simulink model "solar_pv_protected_c07_circuit"  (R2026b)
settings: Solver=VariableStepAuto
model workspace (MAT data in the model file):
  candidate_owner = 'pv_protection_integration_20261023_r01'
  solar_edit_metadata : object (value not decoded)
libraries: fl_lib x149, ee_lib x16, ltc4364demo_lib x3, batteryecm_lib x1, solarprotect_lib x1
(part 15 of 16)

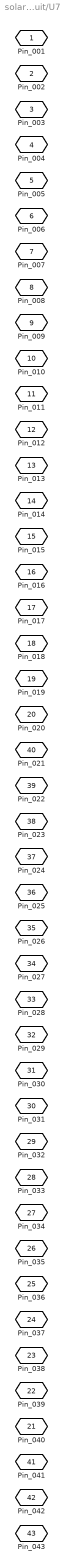
== system solar_pv_protected_c07_circuit/U7 ==
  Pin_001 : PMIOPort  Description=|  Side=Left  ConnectionType=Connection: foundation.electrical.electrical
      | 識別名　　　　　　　; Pin_001
      | 種別　　　　　　　　; Simscape Connection Port（階層境界の物理端子）
      | 所属部品　　　　　　; U7
      | 配置目的　　　　　　; 内部の電気ノードを、この外箱の外側の対応端子へ引き出す。
      | 対応端子　　　　　　; lconn:1／1番 GP0
      | 接続ラベル　　　　　; ラベルなし。接続は実線と境界対応で定義する。
      | モデルの範囲　　　　; 実部品を1個追加する表現ではない。端子自体に増幅・遮断・測定機能を持たない。
      | 端子番号の注意　　　; Connection Portの番号は外箱内の対応番号であり、実パッケージのピン番号とは区別する。
      | 確認の範囲　　　　　; 実ポートと階層対応による静的接続の説明。電気特性の再現性は所属部品の説明を参照する。
      | 
      | 従来の補足　　　　　; 以前のDescriptionを以下に保持する。
      | Physical U7 pin 1 / GP0
      | 
      | 【この説明欄の略語・記号】
      | 用語1　　　　　　　 ; GPIO：General-Purpose Input/Output（汎用入出力端子）。入力・出力や周辺機能に割り当てられる端子。GPの後の数字はRP2040の端子信号番号で、基板上の物理ピン番号とは別。
  Pin_002 : PMIOPort  Description=|  Port=2  Side=Left  ConnectionType=Connection: foundation.electrical.electrical
      | 識別名　　　　　　　; Pin_002
      | 種別　　　　　　　　; Simscape Connection Port（階層境界の物理端子）
      | 所属部品　　　　　　; U7
      | 配置目的　　　　　　; 内部の電気ノードを、この外箱の外側の対応端子へ引き出す。
      | 対応端子　　　　　　; lconn:2／2番 GP1
      | 接続ラベル　　　　　; ラベルなし。接続は実線と境界対応で定義する。
      | モデルの範囲　　　　; 実部品を1個追加する表現ではない。端子自体に増幅・遮断・測定機能を持たない。
      | 端子番号の注意　　　; Connection Portの番号は外箱内の対応番号であり、実パッケージのピン番号とは区別する。
      | 確認の範囲　　　　　; 実ポートと階層対応による静的接続の説明。電気特性の再現性は所属部品の説明を参照する。
      | 
      | 従来の補足　　　　　; 以前のDescriptionを以下に保持する。
      | Physical U7 pin 2 / GP1
      | 
      | 【この説明欄の略語・記号】
      | 用語1　　　　　　　 ; GPIO：General-Purpose Input/Output（汎用入出力端子）。入力・出力や周辺機能に割り当てられる端子。GPの後の数字はRP2040の端子信号番号で、基板上の物理ピン番号とは別。
  Pin_003 : PMIOPort  Description=|  Port=3  Side=Left  ConnectionType=Connection: foundation.electrical.electrical
      | 識別名　　　　　　　; Pin_003
      | 種別　　　　　　　　; Simscape Connection Port（階層境界の物理端子）
      | 所属部品　　　　　　; U7
      | 配置目的　　　　　　; 内部の電気ノードを、この外箱の外側の対応端子へ引き出す。
      | 対応端子　　　　　　; lconn:3／3番 GND
      | 接続ラベル　　　　　; GND、PROT_RETURN
      | モデルの範囲　　　　; 実部品を1個追加する表現ではない。端子自体に増幅・遮断・測定機能を持たない。
      | 端子番号の注意　　　; Connection Portの番号は外箱内の対応番号であり、実パッケージのピン番号とは区別する。
      | 確認の範囲　　　　　; 実ポートと階層対応による静的接続の説明。電気特性の再現性は所属部品の説明を参照する。
      | 
      | 従来の補足　　　　　; 以前のDescriptionを以下に保持する。
      | Physical U7 pin 3 / GND
      | 
      | 【この説明欄の略語・記号】
      | 用語1　　　　　　　 ; GND：Ground（回路の基準電位・電流帰路）。この図の共通基準。保護接地や大地への接続を意味するとは限らない。
      | 用語2　　　　　　　 ; PROT_RETURN：保護回路の共通帰路。PROTはProtection（保護）、RETURNは帰路。プロトタイプの略ではなく、現回路では共通GNDへつながる。
  Pin_004 : PMIOPort  Description=|  Port=4  Side=Left  ConnectionType=Connection: foundation.electrical.electrical
      | 識別名　　　　　　　; Pin_004
      | 種別　　　　　　　　; Simscape Connection Port（階層境界の物理端子）
      | 所属部品　　　　　　; U7
      | 配置目的　　　　　　; 内部の電気ノードを、この外箱の外側の対応端子へ引き出す。
      | 対応端子　　　　　　; lconn:4／4番 GP2
      | 接続ラベル　　　　　; ラベルなし。接続は実線と境界対応で定義する。
      | モデルの範囲　　　　; 実部品を1個追加する表現ではない。端子自体に増幅・遮断・測定機能を持たない。
      | 端子番号の注意　　　; Connection Portの番号は外箱内の対応番号であり、実パッケージのピン番号とは区別する。
      | 確認の範囲　　　　　; 実ポートと階層対応による静的接続の説明。電気特性の再現性は所属部品の説明を参照する。
      | 
      | 従来の補足　　　　　; 以前のDescriptionを以下に保持する。
      | Physical U7 pin 4 / GP2
      | 
      | 【この説明欄の略語・記号】
      | 用語1　　　　　　　 ; GPIO：General-Purpose Input/Output（汎用入出力端子）。入力・出力や周辺機能に割り当てられる端子。GPの後の数字はRP2040の端子信号番号で、基板上の物理ピン番号とは別。
  Pin_005 : PMIOPort  Description=|  Port=5  Side=Left  ConnectionType=Connection: foundation.electrical.electrical
      | 識別名　　　　　　　; Pin_005
      | 種別　　　　　　　　; Simscape Connection Port（階層境界の物理端子）
      | 所属部品　　　　　　; U7
      | 配置目的　　　　　　; 内部の電気ノードを、この外箱の外側の対応端子へ引き出す。
      | 対応端子　　　　　　; lconn:5／5番 GP3
      | 接続ラベル　　　　　; ラベルなし。接続は実線と境界対応で定義する。
      | モデルの範囲　　　　; 実部品を1個追加する表現ではない。端子自体に増幅・遮断・測定機能を持たない。
      | 端子番号の注意　　　; Connection Portの番号は外箱内の対応番号であり、実パッケージのピン番号とは区別する。
      | 確認の範囲　　　　　; 実ポートと階層対応による静的接続の説明。電気特性の再現性は所属部品の説明を参照する。
      | 
      | 従来の補足　　　　　; 以前のDescriptionを以下に保持する。
      | Physical U7 pin 5 / GP3
      | 
      | 【この説明欄の略語・記号】
      | 用語1　　　　　　　 ; GPIO：General-Purpose Input/Output（汎用入出力端子）。入力・出力や周辺機能に割り当てられる端子。GPの後の数字はRP2040の端子信号番号で、基板上の物理ピン番号とは別。
  Pin_006 : PMIOPort  Description=|  Port=6  Side=Left  ConnectionType=Connection: foundation.electrical.electrical
      | 識別名　　　　　　　; Pin_006
      | 種別　　　　　　　　; Simscape Connection Port（階層境界の物理端子）
      | 所属部品　　　　　　; U7
      | 配置目的　　　　　　; 内部の電気ノードを、この外箱の外側の対応端子へ引き出す。
      | 対応端子　　　　　　; lconn:6／6番 GP4
      | 接続ラベル　　　　　; ラベルなし。接続は実線と境界対応で定義する。
      | モデルの範囲　　　　; 実部品を1個追加する表現ではない。端子自体に増幅・遮断・測定機能を持たない。
      | 端子番号の注意　　　; Connection Portの番号は外箱内の対応番号であり、実パッケージのピン番号とは区別する。
      | 確認の範囲　　　　　; 実ポートと階層対応による静的接続の説明。電気特性の再現性は所属部品の説明を参照する。
      | 
      | 従来の補足　　　　　; 以前のDescriptionを以下に保持する。
      | Physical U7 pin 6 / GP4
      | 
      | 【この説明欄の略語・記号】
      | 用語1　　　　　　　 ; GPIO：General-Purpose Input/Output（汎用入出力端子）。入力・出力や周辺機能に割り当てられる端子。GPの後の数字はRP2040の端子信号番号で、基板上の物理ピン番号とは別。
  Pin_007 : PMIOPort  Description=|  Port=7  Side=Left  ConnectionType=Connection: foundation.electrical.electrical
      | 識別名　　　　　　　; Pin_007
      | 種別　　　　　　　　; Simscape Connection Port（階層境界の物理端子）
      | 所属部品　　　　　　; U7
      | 配置目的　　　　　　; 内部の電気ノードを、この外箱の外側の対応端子へ引き出す。
      | 対応端子　　　　　　; lconn:7／7番 GP5
      | 接続ラベル　　　　　; ラベルなし。接続は実線と境界対応で定義する。
      | モデルの範囲　　　　; 実部品を1個追加する表現ではない。端子自体に増幅・遮断・測定機能を持たない。
      | 端子番号の注意　　　; Connection Portの番号は外箱内の対応番号であり、実パッケージのピン番号とは区別する。
      | 確認の範囲　　　　　; 実ポートと階層対応による静的接続の説明。電気特性の再現性は所属部品の説明を参照する。
      | 
      | 従来の補足　　　　　; 以前のDescriptionを以下に保持する。
      | Physical U7 pin 7 / GP5
      | 
      | 【この説明欄の略語・記号】
      | 用語1　　　　　　　 ; GPIO：General-Purpose Input/Output（汎用入出力端子）。入力・出力や周辺機能に割り当てられる端子。GPの後の数字はRP2040の端子信号番号で、基板上の物理ピン番号とは別。
  Pin_008 : PMIOPort  Description=|  Port=8  Side=Left  ConnectionType=Connection: foundation.electrical.electrical
      | 識別名　　　　　　　; Pin_008
      | 種別　　　　　　　　; Simscape Connection Port（階層境界の物理端子）
      | 所属部品　　　　　　; U7
      | 配置目的　　　　　　; 内部の電気ノードを、この外箱の外側の対応端子へ引き出す。
      | 対応端子　　　　　　; lconn:8／8番 GND
      | 接続ラベル　　　　　; GND、PROT_RETURN
      | モデルの範囲　　　　; 実部品を1個追加する表現ではない。端子自体に増幅・遮断・測定機能を持たない。
      | 端子番号の注意　　　; Connection Portの番号は外箱内の対応番号であり、実パッケージのピン番号とは区別する。
      | 確認の範囲　　　　　; 実ポートと階層対応による静的接続の説明。電気特性の再現性は所属部品の説明を参照する。
      | 
      | 従来の補足　　　　　; 以前のDescriptionを以下に保持する。
      | Physical U7 pin 8 / GND
      | 
      | 【この説明欄の略語・記号】
      | 用語1　　　　　　　 ; GND：Ground（回路の基準電位・電流帰路）。この図の共通基準。保護接地や大地への接続を意味するとは限らない。
      | 用語2　　　　　　　 ; PROT_RETURN：保護回路の共通帰路。PROTはProtection（保護）、RETURNは帰路。プロトタイプの略ではなく、現回路では共通GNDへつながる。
  Pin_009 : PMIOPort  Description=|  Port=9  Side=Left  ConnectionType=Connection: foundation.electrical.electrical
      | 識別名　　　　　　　; Pin_009
      | 種別　　　　　　　　; Simscape Connection Port（階層境界の物理端子）
      | 所属部品　　　　　　; U7
      | 配置目的　　　　　　; 内部の電気ノードを、この外箱の外側の対応端子へ引き出す。
      | 対応端子　　　　　　; lconn:9／9番 GP6
      | 接続ラベル　　　　　; GP6
      | モデルの範囲　　　　; 実部品を1個追加する表現ではない。端子自体に増幅・遮断・測定機能を持たない。
      | 端子番号の注意　　　; Connection Portの番号は外箱内の対応番号であり、実パッケージのピン番号とは区別する。
      | 確認の範囲　　　　　; 実ポートと階層対応による静的接続の説明。電気特性の再現性は所属部品の説明を参照する。
      | 
      | 従来の補足　　　　　; 以前のDescriptionを以下に保持する。
      | Physical U7 pin 9 / GP6
      | 
      | 【この説明欄の略語・記号】
      | 用語1　　　　　　　 ; GPIO：General-Purpose Input/Output（汎用入出力端子）。入力・出力や周辺機能に割り当てられる端子。GPの後の数字はRP2040の端子信号番号で、基板上の物理ピン番号とは別。
  Pin_010 : PMIOPort  Description=|  Port=10  Side=Left  ConnectionType=Connection: foundation.electrical.electrical
      | 識別名　　　　　　　; Pin_010
      | 種別　　　　　　　　; Simscape Connection Port（階層境界の物理端子）
      | 所属部品　　　　　　; U7
      | 配置目的　　　　　　; 内部の電気ノードを、この外箱の外側の対応端子へ引き出す。
      | 対応端子　　　　　　; lconn:10／10番 GP7
      | 接続ラベル　　　　　; GP7
      | モデルの範囲　　　　; 実部品を1個追加する表現ではない。端子自体に増幅・遮断・測定機能を持たない。
      | 端子番号の注意　　　; Connection Portの番号は外箱内の対応番号であり、実パッケージのピン番号とは区別する。
      | 確認の範囲　　　　　; 実ポートと階層対応による静的接続の説明。電気特性の再現性は所属部品の説明を参照する。
      | 
      | 従来の補足　　　　　; 以前のDescriptionを以下に保持する。
      | Physical U7 pin 10 / GP7
      | 
      | 【この説明欄の略語・記号】
      | 用語1　　　　　　　 ; GPIO：General-Purpose Input/Output（汎用入出力端子）。入力・出力や周辺機能に割り当てられる端子。GPの後の数字はRP2040の端子信号番号で、基板上の物理ピン番号とは別。
  Pin_011 : PMIOPort  Description=|  Port=11  Side=Left  ConnectionType=Connection: foundation.electrical.electrical
      | 識別名　　　　　　　; Pin_011
      | 種別　　　　　　　　; Simscape Connection Port（階層境界の物理端子）
      | 所属部品　　　　　　; U7
      | 配置目的　　　　　　; 内部の電気ノードを、この外箱の外側の対応端子へ引き出す。
      | 対応端子　　　　　　; lconn:11／11番 GP8
      | 接続ラベル　　　　　; BIAS_EN
      | モデルの範囲　　　　; 実部品を1個追加する表現ではない。端子自体に増幅・遮断・測定機能を持たない。
      | 端子番号の注意　　　; Connection Portの番号は外箱内の対応番号であり、実パッケージのピン番号とは区別する。
      | 確認の範囲　　　　　; 実ポートと階層対応による静的接続の説明。電気特性の再現性は所属部品の説明を参照する。
      | 
      | 従来の補足　　　　　; 以前のDescriptionを以下に保持する。
      | Physical U7 pin 11 / GP8
      | 
      | 【この説明欄の略語・記号】
      | 用語1　　　　　　　 ; GPIO：General-Purpose Input/Output（汎用入出力端子）。入力・出力や周辺機能に割り当てられる端子。GPの後の数字はRP2040の端子信号番号で、基板上の物理ピン番号とは別。
      | 用語2　　　　　　　 ; EN：Enable（動作許可）。対象機能の動作を許可する信号。端子ごとの有効レベルや接続状態に従う。
  Pin_012 : PMIOPort  Description=|  Port=12  Side=Left  ConnectionType=Connection: foundation.electrical.electrical
      | 識別名　　　　　　　; Pin_012
      | 種別　　　　　　　　; Simscape Connection Port（階層境界の物理端子）
      | 所属部品　　　　　　; U7
      | 配置目的　　　　　　; 内部の電気ノードを、この外箱の外側の対応端子へ引き出す。
      | 対応端子　　　　　　; lconn:12／12番 GP9
      | 接続ラベル　　　　　; BIAS_PG
      | モデルの範囲　　　　; 実部品を1個追加する表現ではない。端子自体に増幅・遮断・測定機能を持たない。
      | 端子番号の注意　　　; Connection Portの番号は外箱内の対応番号であり、実パッケージのピン番号とは区別する。
      | 確認の範囲　　　　　; 実ポートと階層対応による静的接続の説明。電気特性の再現性は所属部品の説明を参照する。
      | 
      | 従来の補足　　　　　; 以前のDescriptionを以下に保持する。
      | Physical U7 pin 12 / GP9
      | 
      | 【この説明欄の略語・記号】
      | 用語1　　　　　　　 ; IC：Integrated Circuit（集積回路）。複数の電子素子と機能を小さな半導体チップに集積した部品。
      | 用語2　　　　　　　 ; GPIO：General-Purpose Input/Output（汎用入出力端子）。入力・出力や周辺機能に割り当てられる端子。GPの後の数字はRP2040の端子信号番号で、基板上の物理ピン番号とは別。
      | 用語3　　　　　　　 ; PG：Power Good（電源状態通知）。電源出力が規定状態にあるかを知らせる信号。プルアップ条件と実際の通知条件は対象ICの説明で確認する。
  Pin_013 : PMIOPort  Description=|  Port=13  Side=Left  ConnectionType=Connection: foundation.electrical.electrical
      | 識別名　　　　　　　; Pin_013
      | 種別　　　　　　　　; Simscape Connection Port（階層境界の物理端子）
      | 所属部品　　　　　　; U7
      | 配置目的　　　　　　; 内部の電気ノードを、この外箱の外側の対応端子へ引き出す。
      | 対応端子　　　　　　; lconn:13／13番 GND
      | 接続ラベル　　　　　; GND、PROT_RETURN
      | モデルの範囲　　　　; 実部品を1個追加する表現ではない。端子自体に増幅・遮断・測定機能を持たない。
      | 端子番号の注意　　　; Connection Portの番号は外箱内の対応番号であり、実パッケージのピン番号とは区別する。
      | 確認の範囲　　　　　; 実ポートと階層対応による静的接続の説明。電気特性の再現性は所属部品の説明を参照する。
      | 
      | 従来の補足　　　　　; 以前のDescriptionを以下に保持する。
      | Physical U7 pin 13 / GND
      | 
      | 【この説明欄の略語・記号】
      | 用語1　　　　　　　 ; GND：Ground（回路の基準電位・電流帰路）。この図の共通基準。保護接地や大地への接続を意味するとは限らない。
      | 用語2　　　　　　　 ; PROT_RETURN：保護回路の共通帰路。PROTはProtection（保護）、RETURNは帰路。プロトタイプの略ではなく、現回路では共通GNDへつながる。
  Pin_014 : PMIOPort  Description=|  Port=14  Side=Left  ConnectionType=Connection: foundation.electrical.electrical
      | 識別名　　　　　　　; Pin_014
      | 種別　　　　　　　　; Simscape Connection Port（階層境界の物理端子）
      | 所属部品　　　　　　; U7
      | 配置目的　　　　　　; 内部の電気ノードを、この外箱の外側の対応端子へ引き出す。
      | 対応端子　　　　　　; lconn:14／14番 GP10
      | 接続ラベル　　　　　; ラベルなし。接続は実線と境界対応で定義する。
      | モデルの範囲　　　　; 実部品を1個追加する表現ではない。端子自体に増幅・遮断・測定機能を持たない。
      | 端子番号の注意　　　; Connection Portの番号は外箱内の対応番号であり、実パッケージのピン番号とは区別する。
      | 確認の範囲　　　　　; 実ポートと階層対応による静的接続の説明。電気特性の再現性は所属部品の説明を参照する。
      | 
      | 従来の補足　　　　　; 以前のDescriptionを以下に保持する。
      | Physical U7 pin 14 / GP10
      | 
      | 【この説明欄の略語・記号】
      | 用語1　　　　　　　 ; GPIO：General-Purpose Input/Output（汎用入出力端子）。入力・出力や周辺機能に割り当てられる端子。GPの後の数字はRP2040の端子信号番号で、基板上の物理ピン番号とは別。
  Pin_015 : PMIOPort  Description=|  Port=15  Side=Left  ConnectionType=Connection: foundation.electrical.electrical
      | 識別名　　　　　　　; Pin_015
      | 種別　　　　　　　　; Simscape Connection Port（階層境界の物理端子）
      | 所属部品　　　　　　; U7
      | 配置目的　　　　　　; 内部の電気ノードを、この外箱の外側の対応端子へ引き出す。
      | 対応端子　　　　　　; lconn:15／15番 GP11
      | 接続ラベル　　　　　; MAIN_EN
      | モデルの範囲　　　　; 実部品を1個追加する表現ではない。端子自体に増幅・遮断・測定機能を持たない。
      | 端子番号の注意　　　; Connection Portの番号は外箱内の対応番号であり、実パッケージのピン番号とは区別する。
      | 確認の範囲　　　　　; 実ポートと階層対応による静的接続の説明。電気特性の再現性は所属部品の説明を参照する。
      | 
      | 従来の補足　　　　　; 以前のDescriptionを以下に保持する。
      | Physical U7 pin 15 / GP11
      | 
      | 【この説明欄の略語・記号】
      | 用語1　　　　　　　 ; GPIO：General-Purpose Input/Output（汎用入出力端子）。入力・出力や周辺機能に割り当てられる端子。GPの後の数字はRP2040の端子信号番号で、基板上の物理ピン番号とは別。
      | 用語2　　　　　　　 ; EN：Enable（動作許可）。対象機能の動作を許可する信号。端子ごとの有効レベルや接続状態に従う。
  Pin_016 : PMIOPort  Description=|  Port=16  Side=Left  ConnectionType=Connection: foundation.electrical.electrical
      | 識別名　　　　　　　; Pin_016
      | 種別　　　　　　　　; Simscape Connection Port（階層境界の物理端子）
      | 所属部品　　　　　　; U7
      | 配置目的　　　　　　; 内部の電気ノードを、この外箱の外側の対応端子へ引き出す。
      | 対応端子　　　　　　; lconn:16／16番 GP12
      | 接続ラベル　　　　　; ラベルなし。接続は実線と境界対応で定義する。
      | モデルの範囲　　　　; 実部品を1個追加する表現ではない。端子自体に増幅・遮断・測定機能を持たない。
      | 端子番号の注意　　　; Connection Portの番号は外箱内の対応番号であり、実パッケージのピン番号とは区別する。
      | 確認の範囲　　　　　; 実ポートと階層対応による静的接続の説明。電気特性の再現性は所属部品の説明を参照する。
      | 
      | 従来の補足　　　　　; 以前のDescriptionを以下に保持する。
      | Physical U7 pin 16 / GP12
      | 
      | 【この説明欄の略語・記号】
      | 用語1　　　　　　　 ; GPIO：General-Purpose Input/Output（汎用入出力端子）。入力・出力や周辺機能に割り当てられる端子。GPの後の数字はRP2040の端子信号番号で、基板上の物理ピン番号とは別。
  Pin_017 : PMIOPort  Description=|  Port=17  Side=Left  ConnectionType=Connection: foundation.electrical.electrical
      | 識別名　　　　　　　; Pin_017
      | 種別　　　　　　　　; Simscape Connection Port（階層境界の物理端子）
      | 所属部品　　　　　　; U7
      | 配置目的　　　　　　; 内部の電気ノードを、この外箱の外側の対応端子へ引き出す。
      | 対応端子　　　　　　; lconn:17／17番 GP13
      | 接続ラベル　　　　　; PROTECTION_FLT_N
      | モデルの範囲　　　　; 実部品を1個追加する表現ではない。端子自体に増幅・遮断・測定機能を持たない。
      | 端子番号の注意　　　; Connection Portの番号は外箱内の対応番号であり、実パッケージのピン番号とは区別する。
      | 確認の範囲　　　　　; 実ポートと階層対応による静的接続の説明。電気特性の再現性は所属部品の説明を参照する。
      | 
      | 従来の補足　　　　　; 以前のDescriptionを以下に保持する。
      | Physical U7 pin 17 / GP13
      | 
      | 【この説明欄の略語・記号】
      | 用語1　　　　　　　 ; GPIO：General-Purpose Input/Output（汎用入出力端子）。入力・出力や周辺機能に割り当てられる端子。GPの後の数字はRP2040の端子信号番号で、基板上の物理ピン番号とは別。
      | 用語2　　　　　　　 ; FLT：Fault（故障状態通知）。LTC4364の故障警告出力。全種類の異常や逆流を一律に通知する信号という意味ではない。
  Pin_018 : PMIOPort  Description=|  Port=18  Side=Left  ConnectionType=Connection: foundation.electrical.electrical
      | 識別名　　　　　　　; Pin_018
      | 種別　　　　　　　　; Simscape Connection Port（階層境界の物理端子）
      | 所属部品　　　　　　; U7
      | 配置目的　　　　　　; 内部の電気ノードを、この外箱の外側の対応端子へ引き出す。
      | 対応端子　　　　　　; lconn:18／18番 GND
      | 接続ラベル　　　　　; GND、PROT_RETURN
      | モデルの範囲　　　　; 実部品を1個追加する表現ではない。端子自体に増幅・遮断・測定機能を持たない。
      | 端子番号の注意　　　; Connection Portの番号は外箱内の対応番号であり、実パッケージのピン番号とは区別する。
      | 確認の範囲　　　　　; 実ポートと階層対応による静的接続の説明。電気特性の再現性は所属部品の説明を参照する。
      | 
      | 従来の補足　　　　　; 以前のDescriptionを以下に保持する。
      | Physical U7 pin 18 / GND
      | 
      | 【この説明欄の略語・記号】
      | 用語1　　　　　　　 ; GND：Ground（回路の基準電位・電流帰路）。この図の共通基準。保護接地や大地への接続を意味するとは限らない。
      | 用語2　　　　　　　 ; PROT_RETURN：保護回路の共通帰路。PROTはProtection（保護）、RETURNは帰路。プロトタイプの略ではなく、現回路では共通GNDへつながる。
  Pin_019 : PMIOPort  Description=|  Port=19  Side=Left  ConnectionType=Connection: foundation.electrical.electrical
      | 識別名　　　　　　　; Pin_019
      | 種別　　　　　　　　; Simscape Connection Port（階層境界の物理端子）
      | 所属部品　　　　　　; U7
      | 配置目的　　　　　　; 内部の電気ノードを、この外箱の外側の対応端子へ引き出す。
      | 対応端子　　　　　　; lconn:19／19番 GP14
      | 接続ラベル　　　　　; ラベルなし。接続は実線と境界対応で定義する。
      | モデルの範囲　　　　; 実部品を1個追加する表現ではない。端子自体に増幅・遮断・測定機能を持たない。
      | 端子番号の注意　　　; Connection Portの番号は外箱内の対応番号であり、実パッケージのピン番号とは区別する。
      | 確認の範囲　　　　　; 実ポートと階層対応による静的接続の説明。電気特性の再現性は所属部品の説明を参照する。
      | 
      | 従来の補足　　　　　; 以前のDescriptionを以下に保持する。
      | Physical U7 pin 19 / GP14
      | 
      | 【この説明欄の略語・記号】
      | 用語1　　　　　　　 ; GPIO：General-Purpose Input/Output（汎用入出力端子）。入力・出力や周辺機能に割り当てられる端子。GPの後の数字はRP2040の端子信号番号で、基板上の物理ピン番号とは別。
  Pin_020 : PMIOPort  Description=|  Port=20  Side=Left  ConnectionType=Connection: foundation.electrical.electrical
      | 識別名　　　　　　　; Pin_020
      | 種別　　　　　　　　; Simscape Connection Port（階層境界の物理端子）
      | 所属部品　　　　　　; U7
      | 配置目的　　　　　　; 内部の電気ノードを、この外箱の外側の対応端子へ引き出す。
      | 対応端子　　　　　　; lconn:20／20番 GP15
      | 接続ラベル　　　　　; ラベルなし。接続は実線と境界対応で定義する。
      | モデルの範囲　　　　; 実部品を1個追加する表現ではない。端子自体に増幅・遮断・測定機能を持たない。
      | 端子番号の注意　　　; Connection Portの番号は外箱内の対応番号であり、実パッケージのピン番号とは区別する。
      | 確認の範囲　　　　　; 実ポートと階層対応による静的接続の説明。電気特性の再現性は所属部品の説明を参照する。
      | 
      | 従来の補足　　　　　; 以前のDescriptionを以下に保持する。
      | Physical U7 pin 20 / GP15
      | 
      | 【この説明欄の略語・記号】
      | 用語1　　　　　　　 ; GPIO：General-Purpose Input/Output（汎用入出力端子）。入力・出力や周辺機能に割り当てられる端子。GPの後の数字はRP2040の端子信号番号で、基板上の物理ピン番号とは別。
  Pin_040 : PMIOPort  Description=|  Port=21  Side=Right  ConnectionType=Connection: foundation.electrical.electrical
      | 識別名　　　　　　　; Pin_040
      | 種別　　　　　　　　; Simscape Connection Port（階層境界の物理端子）
      | 所属部品　　　　　　; U7
      | 配置目的　　　　　　; 内部の電気ノードを、この外箱の外側の対応端子へ引き出す。
      | 対応端子　　　　　　; rconn:20／40番 VBUS
      | 接続ラベル　　　　　; ラベルなし。接続は実線と境界対応で定義する。
      | モデルの範囲　　　　; 実部品を1個追加する表現ではない。端子自体に増幅・遮断・測定機能を持たない。
      | 端子番号の注意　　　; Connection Portの番号は外箱内の対応番号であり、実パッケージのピン番号とは区別する。
      | 確認の範囲　　　　　; 実ポートと階層対応による静的接続の説明。電気特性の再現性は所属部品の説明を参照する。
      | 
      | 従来の補足　　　　　; 以前のDescriptionを以下に保持する。
      | Physical U7 pin 40 / VBUS
  Pin_039 : PMIOPort  Description=|  Port=22  Side=Right  ConnectionType=Connection: foundation.electrical.electrical
      | 識別名　　　　　　　; Pin_039
      | 種別　　　　　　　　; Simscape Connection Port（階層境界の物理端子）
      | 所属部品　　　　　　; U7
      | 配置目的　　　　　　; 内部の電気ノードを、この外箱の外側の対応端子へ引き出す。
      | 対応端子　　　　　　; rconn:19／39番 VSYS
      | 接続ラベル　　　　　; VSYS_5V
      | モデルの範囲　　　　; 実部品を1個追加する表現ではない。端子自体に増幅・遮断・測定機能を持たない。
      | 端子番号の注意　　　; Connection Portの番号は外箱内の対応番号であり、実パッケージのピン番号とは区別する。
      | 確認の範囲　　　　　; 実ポートと階層対応による静的接続の説明。電気特性の再現性は所属部品の説明を参照する。
      | 
      | 従来の補足　　　　　; 以前のDescriptionを以下に保持する。
      | Physical U7 pin 39 / VSYS
  Pin_038 : PMIOPort  Description=|  Port=23  Side=Right  ConnectionType=Connection: foundation.electrical.electrical
      | 識別名　　　　　　　; Pin_038
      | 種別　　　　　　　　; Simscape Connection Port（階層境界の物理端子）
      | 所属部品　　　　　　; U7
      | 配置目的　　　　　　; 内部の電気ノードを、この外箱の外側の対応端子へ引き出す。
      | 対応端子　　　　　　; rconn:18／38番 GND
      | 接続ラベル　　　　　; GND、PROT_RETURN
      | モデルの範囲　　　　; 実部品を1個追加する表現ではない。端子自体に増幅・遮断・測定機能を持たない。
      | 端子番号の注意　　　; Connection Portの番号は外箱内の対応番号であり、実パッケージのピン番号とは区別する。
      | 確認の範囲　　　　　; 実ポートと階層対応による静的接続の説明。電気特性の再現性は所属部品の説明を参照する。
      | 
      | 従来の補足　　　　　; 以前のDescriptionを以下に保持する。
      | Physical U7 pin 38 / GND
      | 
      | 【この説明欄の略語・記号】
      | 用語1　　　　　　　 ; GND：Ground（回路の基準電位・電流帰路）。この図の共通基準。保護接地や大地への接続を意味するとは限らない。
      | 用語2　　　　　　　 ; PROT_RETURN：保護回路の共通帰路。PROTはProtection（保護）、RETURNは帰路。プロトタイプの略ではなく、現回路では共通GNDへつながる。
  Pin_037 : PMIOPort  Description=|  Port=24  Side=Right  ConnectionType=Connection: foundation.electrical.electrical
      | 識別名　　　　　　　; Pin_037
      | 種別　　　　　　　　; Simscape Connection Port（階層境界の物理端子）
      | 所属部品　　　　　　; U7
      | 配置目的　　　　　　; 内部の電気ノードを、この外箱の外側の対応端子へ引き出す。
      | 対応端子　　　　　　; rconn:17／37番 3V3_EN
      | 接続ラベル　　　　　; ラベルなし。接続は実線と境界対応で定義する。
      | モデルの範囲　　　　; 実部品を1個追加する表現ではない。端子自体に増幅・遮断・測定機能を持たない。
      | 端子番号の注意　　　; Connection Portの番号は外箱内の対応番号であり、実パッケージのピン番号とは区別する。
      | 確認の範囲　　　　　; 実ポートと階層対応による静的接続の説明。電気特性の再現性は所属部品の説明を参照する。
      | 
      | 従来の補足　　　　　; 以前のDescriptionを以下に保持する。
      | Physical U7 pin 37 / 3V3_EN
      | 
      | 【この説明欄の略語・記号】
      | 用語1　　　　　　　 ; EN：Enable（動作許可）。対象機能の動作を許可する信号。端子ごとの有効レベルや接続状態に従う。
  Pin_036 : PMIOPort  Description=|  Port=25  Side=Right  ConnectionType=Connection: foundation.electrical.electrical
      | 識別名　　　　　　　; Pin_036
      | 種別　　　　　　　　; Simscape Connection Port（階層境界の物理端子）
      | 所属部品　　　　　　; U7
      | 配置目的　　　　　　; 内部の電気ノードを、この外箱の外側の対応端子へ引き出す。
      | 対応端子　　　　　　; rconn:16／36番 3V3_OUT
      | 接続ラベル　　　　　; V3V3
      | モデルの範囲　　　　; 実部品を1個追加する表現ではない。端子自体に増幅・遮断・測定機能を持たない。
      | 端子番号の注意　　　; Connection Portの番号は外箱内の対応番号であり、実パッケージのピン番号とは区別する。
      | 確認の範囲　　　　　; 実ポートと階層対応による静的接続の説明。電気特性の再現性は所属部品の説明を参照する。
      | 
      | 従来の補足　　　　　; 以前のDescriptionを以下に保持する。
      | Physical U7 pin 36 / 3V3_OUT
  Pin_035 : PMIOPort  Description=|  Port=26  Side=Right  ConnectionType=Connection: foundation.electrical.electrical
      | 識別名　　　　　　　; Pin_035
      | 種別　　　　　　　　; Simscape Connection Port（階層境界の物理端子）
      | 所属部品　　　　　　; U7
      | 配置目的　　　　　　; 内部の電気ノードを、この外箱の外側の対応端子へ引き出す。
      | 対応端子　　　　　　; rconn:15／35番 ADC_VREF
      | 接続ラベル　　　　　; ラベルなし。接続は実線と境界対応で定義する。
      | モデルの範囲　　　　; 実部品を1個追加する表現ではない。端子自体に増幅・遮断・測定機能を持たない。
      | 端子番号の注意　　　; Connection Portの番号は外箱内の対応番号であり、実パッケージのピン番号とは区別する。
      | 確認の範囲　　　　　; 実ポートと階層対応による静的接続の説明。電気特性の再現性は所属部品の説明を参照する。
      | 
      | 従来の補足　　　　　; 以前のDescriptionを以下に保持する。
      | Physical U7 pin 35 / ADC_VREF
      | 
      | 【この説明欄の略語・記号】
      | 用語1　　　　　　　 ; ADC：Analog-to-Digital Converter（アナログ・デジタル変換器）。測定電圧をデジタル値へ変換する回路。電流や温度も、センサーで電圧へ変換した後に読み取る。
      | 用語2　　　　　　　 ; VREF/REF：基準電圧を表す端子名。REFはReference（基準）の意味。ADCの変換尺度や電流アンプの出力基準に使う。REF1/REF2の接続電位は個別に確認する。
  Pin_034 : PMIOPort  Description=|  Port=27  Side=Right  ConnectionType=Connection: foundation.electrical.electrical
      | 識別名　　　　　　　; Pin_034
      | 種別　　　　　　　　; Simscape Connection Port（階層境界の物理端子）
      | 所属部品　　　　　　; U7
      | 配置目的　　　　　　; 内部の電気ノードを、この外箱の外側の対応端子へ引き出す。
      | 対応端子　　　　　　; rconn:14／34番 GP28
      | 接続ラベル　　　　　; ラベルなし。接続は実線と境界対応で定義する。
      | モデルの範囲　　　　; 実部品を1個追加する表現ではない。端子自体に増幅・遮断・測定機能を持たない。
      | 端子番号の注意　　　; Connection Portの番号は外箱内の対応番号であり、実パッケージのピン番号とは区別する。
      | 確認の範囲　　　　　; 実ポートと階層対応による静的接続の説明。電気特性の再現性は所属部品の説明を参照する。
      | 
      | 従来の補足　　　　　; 以前のDescriptionを以下に保持する。
      | Physical U7 pin 34 / GP28
      | 
      | 【この説明欄の略語・記号】
      | 用語1　　　　　　　 ; GPIO：General-Purpose Input/Output（汎用入出力端子）。入力・出力や周辺機能に割り当てられる端子。GPの後の数字はRP2040の端子信号番号で、基板上の物理ピン番号とは別。
  Pin_033 : PMIOPort  Description=|  Port=28  Side=Right  ConnectionType=Connection: foundation.electrical.electrical
      | 識別名　　　　　　　; Pin_033
      | 種別　　　　　　　　; Simscape Connection Port（階層境界の物理端子）
      | 所属部品　　　　　　; U7
      | 配置目的　　　　　　; 内部の電気ノードを、この外箱の外側の対応端子へ引き出す。
      | 対応端子　　　　　　; rconn:13／33番 AGND
      | 接続ラベル　　　　　; GND、PROT_RETURN
      | モデルの範囲　　　　; 実部品を1個追加する表現ではない。端子自体に増幅・遮断・測定機能を持たない。
      | 端子番号の注意　　　; Connection Portの番号は外箱内の対応番号であり、実パッケージのピン番号とは区別する。
      | 確認の範囲　　　　　; 実ポートと階層対応による静的接続の説明。電気特性の再現性は所属部品の説明を参照する。
      | 
      | 従来の補足　　　　　; 以前のDescriptionを以下に保持する。
      | Physical U7 pin 33 / AGND
      | 
      | 【この説明欄の略語・記号】
      | 用語1　　　　　　　 ; GND：Ground（回路の基準電位・電流帰路）。この図の共通基準。保護接地や大地への接続を意味するとは限らない。
      | 用語2　　　　　　　 ; AGND：Analog Ground（アナログ回路の基準端子）。アナログ部分の電流帰路。現図では共通GNDへ接続されるが、実装時の電流経路への配慮は別途必要。
      | 用語3　　　　　　　 ; PROT_RETURN：保護回路の共通帰路。PROTはProtection（保護）、RETURNは帰路。プロトタイプの略ではなく、現回路では共通GNDへつながる。
  Pin_032 : PMIOPort  Description=|  Port=29  Side=Right  ConnectionType=Connection: foundation.electrical.electrical
      | 識別名　　　　　　　; Pin_032
      | 種別　　　　　　　　; Simscape Connection Port（階層境界の物理端子）
      | 所属部品　　　　　　; U7
      | 配置目的　　　　　　; 内部の電気ノードを、この外箱の外側の対応端子へ引き出す。
      | 対応端子　　　　　　; rconn:12／32番 GP27
      | 接続ラベル　　　　　; ラベルなし。接続は実線と境界対応で定義する。
      | モデルの範囲　　　　; 実部品を1個追加する表現ではない。端子自体に増幅・遮断・測定機能を持たない。
      | 端子番号の注意　　　; Connection Portの番号は外箱内の対応番号であり、実パッケージのピン番号とは区別する。
      | 確認の範囲　　　　　; 実ポートと階層対応による静的接続の説明。電気特性の再現性は所属部品の説明を参照する。
      | 
      | 従来の補足　　　　　; 以前のDescriptionを以下に保持する。
      | Physical U7 pin 32 / GP27
      | 
      | 【この説明欄の略語・記号】
      | 用語1　　　　　　　 ; GPIO：General-Purpose Input/Output（汎用入出力端子）。入力・出力や周辺機能に割り当てられる端子。GPの後の数字はRP2040の端子信号番号で、基板上の物理ピン番号とは別。
  Pin_031 : PMIOPort  Description=|  Port=30  Side=Right  ConnectionType=Connection: foundation.electrical.electrical
      | 識別名　　　　　　　; Pin_031
      | 種別　　　　　　　　; Simscape Connection Port（階層境界の物理端子）
      | 所属部品　　　　　　; U7
      | 配置目的　　　　　　; 内部の電気ノードを、この外箱の外側の対応端子へ引き出す。
      | 対応端子　　　　　　; rconn:11／31番 GP26
      | 接続ラベル　　　　　; ラベルなし。接続は実線と境界対応で定義する。
      | モデルの範囲　　　　; 実部品を1個追加する表現ではない。端子自体に増幅・遮断・測定機能を持たない。
      | 端子番号の注意　　　; Connection Portの番号は外箱内の対応番号であり、実パッケージのピン番号とは区別する。
      | 確認の範囲　　　　　; 実ポートと階層対応による静的接続の説明。電気特性の再現性は所属部品の説明を参照する。
      | 
      | 従来の補足　　　　　; 以前のDescriptionを以下に保持する。
      | Physical U7 pin 31 / GP26
      | 
      | 【この説明欄の略語・記号】
      | 用語1　　　　　　　 ; GPIO：General-Purpose Input/Output（汎用入出力端子）。入力・出力や周辺機能に割り当てられる端子。GPの後の数字はRP2040の端子信号番号で、基板上の物理ピン番号とは別。
  Pin_030 : PMIOPort  Description=|  Port=31  Side=Right  ConnectionType=Connection: foundation.electrical.electrical
      | 識別名　　　　　　　; Pin_030
      | 種別　　　　　　　　; Simscape Connection Port（階層境界の物理端子）
      | 所属部品　　　　　　; U7
      | 配置目的　　　　　　; 内部の電気ノードを、この外箱の外側の対応端子へ引き出す。
      | 対応端子　　　　　　; rconn:10／30番 RUN
      | 接続ラベル　　　　　; ラベルなし。接続は実線と境界対応で定義する。
      | モデルの範囲　　　　; 実部品を1個追加する表現ではない。端子自体に増幅・遮断・測定機能を持たない。
      | 端子番号の注意　　　; Connection Portの番号は外箱内の対応番号であり、実パッケージのピン番号とは区別する。
      | 確認の範囲　　　　　; 実ポートと階層対応による静的接続の説明。電気特性の再現性は所属部品の説明を参照する。
      | 
      | 従来の補足　　　　　; 以前のDescriptionを以下に保持する。
      | Physical U7 pin 30 / RUN
  Pin_029 : PMIOPort  Description=|  Port=32  Side=Right  ConnectionType=Connection: foundation.electrical.electrical
      | 識別名　　　　　　　; Pin_029
      | 種別　　　　　　　　; Simscape Connection Port（階層境界の物理端子）
      | 所属部品　　　　　　; U7
      | 配置目的　　　　　　; 内部の電気ノードを、この外箱の外側の対応端子へ引き出す。
      | 対応端子　　　　　　; rconn:9／29番 GP22
      | 接続ラベル　　　　　; ラベルなし。接続は実線と境界対応で定義する。
      | モデルの範囲　　　　; 実部品を1個追加する表現ではない。端子自体に増幅・遮断・測定機能を持たない。
      | 端子番号の注意　　　; Connection Portの番号は外箱内の対応番号であり、実パッケージのピン番号とは区別する。
      | 確認の範囲　　　　　; 実ポートと階層対応による静的接続の説明。電気特性の再現性は所属部品の説明を参照する。
      | 
      | 従来の補足　　　　　; 以前のDescriptionを以下に保持する。
      | Physical U7 pin 29 / GP22
      | 
      | 【この説明欄の略語・記号】
      | 用語1　　　　　　　 ; GPIO：General-Purpose Input/Output（汎用入出力端子）。入力・出力や周辺機能に割り当てられる端子。GPの後の数字はRP2040の端子信号番号で、基板上の物理ピン番号とは別。
  Pin_028 : PMIOPort  Description=|  Port=33  Side=Right  ConnectionType=Connection: foundation.electrical.electrical
      | 識別名　　　　　　　; Pin_028
      | 種別　　　　　　　　; Simscape Connection Port（階層境界の物理端子）
      | 所属部品　　　　　　; U7
      | 配置目的　　　　　　; 内部の電気ノードを、この外箱の外側の対応端子へ引き出す。
      | 対応端子　　　　　　; rconn:8／28番 GND
      | 接続ラベル　　　　　; GND、PROT_RETURN
      | モデルの範囲　　　　; 実部品を1個追加する表現ではない。端子自体に増幅・遮断・測定機能を持たない。
      | 端子番号の注意　　　; Connection Portの番号は外箱内の対応番号であり、実パッケージのピン番号とは区別する。
      | 確認の範囲　　　　　; 実ポートと階層対応による静的接続の説明。電気特性の再現性は所属部品の説明を参照する。
      | 
      | 従来の補足　　　　　; 以前のDescriptionを以下に保持する。
      | Physical U7 pin 28 / GND
      | 
      | 【この説明欄の略語・記号】
      | 用語1　　　　　　　 ; GND：Ground（回路の基準電位・電流帰路）。この図の共通基準。保護接地や大地への接続を意味するとは限らない。
      | 用語2　　　　　　　 ; PROT_RETURN：保護回路の共通帰路。PROTはProtection（保護）、RETURNは帰路。プロトタイプの略ではなく、現回路では共通GNDへつながる。
  Pin_027 : PMIOPort  Description=|  Port=34  Side=Right  ConnectionType=Connection: foundation.electrical.electrical
      | 識別名　　　　　　　; Pin_027
      | 種別　　　　　　　　; Simscape Connection Port（階層境界の物理端子）
      | 所属部品　　　　　　; U7
      | 配置目的　　　　　　; 内部の電気ノードを、この外箱の外側の対応端子へ引き出す。
      | 対応端子　　　　　　; rconn:7／27番 GP21
      | 接続ラベル　　　　　; ラベルなし。接続は実線と境界対応で定義する。
      | モデルの範囲　　　　; 実部品を1個追加する表現ではない。端子自体に増幅・遮断・測定機能を持たない。
      | 端子番号の注意　　　; Connection Portの番号は外箱内の対応番号であり、実パッケージのピン番号とは区別する。
      | 確認の範囲　　　　　; 実ポートと階層対応による静的接続の説明。電気特性の再現性は所属部品の説明を参照する。
      | 
      | 従来の補足　　　　　; 以前のDescriptionを以下に保持する。
      | Physical U7 pin 27 / GP21
      | 
      | 【この説明欄の略語・記号】
      | 用語1　　　　　　　 ; GPIO：General-Purpose Input/Output（汎用入出力端子）。入力・出力や周辺機能に割り当てられる端子。GPの後の数字はRP2040の端子信号番号で、基板上の物理ピン番号とは別。
  Pin_026 : PMIOPort  Description=|  Port=35  Side=Right  ConnectionType=Connection: foundation.electrical.electrical
      | 識別名　　　　　　　; Pin_026
      | 種別　　　　　　　　; Simscape Connection Port（階層境界の物理端子）
      | 所属部品　　　　　　; U7
      | 配置目的　　　　　　; 内部の電気ノードを、この外箱の外側の対応端子へ引き出す。
      | 対応端子　　　　　　; rconn:6／26番 GP20
      | 接続ラベル　　　　　; ラベルなし。接続は実線と境界対応で定義する。
      | モデルの範囲　　　　; 実部品を1個追加する表現ではない。端子自体に増幅・遮断・測定機能を持たない。
      | 端子番号の注意　　　; Connection Portの番号は外箱内の対応番号であり、実パッケージのピン番号とは区別する。
      | 確認の範囲　　　　　; 実ポートと階層対応による静的接続の説明。電気特性の再現性は所属部品の説明を参照する。
      | 
      | 従来の補足　　　　　; 以前のDescriptionを以下に保持する。
      | Physical U7 pin 26 / GP20
      | 
      | 【この説明欄の略語・記号】
      | 用語1　　　　　　　 ; GPIO：General-Purpose Input/Output（汎用入出力端子）。入力・出力や周辺機能に割り当てられる端子。GPの後の数字はRP2040の端子信号番号で、基板上の物理ピン番号とは別。
  Pin_025 : PMIOPort  Description=|  Port=36  Side=Right  ConnectionType=Connection: foundation.electrical.electrical
      | 識別名　　　　　　　; Pin_025
      | 種別　　　　　　　　; Simscape Connection Port（階層境界の物理端子）
      | 所属部品　　　　　　; U7
      | 配置目的　　　　　　; 内部の電気ノードを、この外箱の外側の対応端子へ引き出す。
      | 対応端子　　　　　　; rconn:5／25番 GP19
      | 接続ラベル　　　　　; SPI_MOSI
      | モデルの範囲　　　　; 実部品を1個追加する表現ではない。端子自体に増幅・遮断・測定機能を持たない。
      | 端子番号の注意　　　; Connection Portの番号は外箱内の対応番号であり、実パッケージのピン番号とは区別する。
      | 確認の範囲　　　　　; 実ポートと階層対応による静的接続の説明。電気特性の再現性は所属部品の説明を参照する。
      | 
      | 従来の補足　　　　　; 以前のDescriptionを以下に保持する。
      | Physical U7 pin 25 / GP19
      | 
      | 【この説明欄の略語・記号】
      | 用語1　　　　　　　 ; ADC：Analog-to-Digital Converter（アナログ・デジタル変換器）。測定電圧をデジタル値へ変換する回路。電流や温度も、センサーで電圧へ変換した後に読み取る。
      | 用語2　　　　　　　 ; GPIO：General-Purpose Input/Output（汎用入出力端子）。入力・出力や周辺機能に割り当てられる端子。GPの後の数字はRP2040の端子信号番号で、基板上の物理ピン番号とは別。
      | 用語3　　　　　　　 ; SPI：Serial Peripheral Interface（同期式シリアル通信）。クロックとデータ線を使う通信方式。本回路ではRP2040と外付け測定用ADCの通信に使う。
      | 用語4　　　　　　　 ; MOSI：Master Out, Slave In（制御側から出るSPIデータ線）。この回路ではRP2040からADCのDINへ測定チャネル選択などの情報が流れる。
      | 用語5　　　　　　　 ; DIN：Data In（データ入力端子）。ADC側から見たデジタルデータ入力。測定対象のアナログ電圧入力とは別。
  Pin_024 : PMIOPort  Description=|  Port=37  Side=Right  ConnectionType=Connection: foundation.electrical.electrical
      | 識別名　　　　　　　; Pin_024
      | 種別　　　　　　　　; Simscape Connection Port（階層境界の物理端子）
      | 所属部品　　　　　　; U7
      | 配置目的　　　　　　; 内部の電気ノードを、この外箱の外側の対応端子へ引き出す。
      | 対応端子　　　　　　; rconn:4／24番 GP18
      | 接続ラベル　　　　　; SPI_SCK
      | モデルの範囲　　　　; 実部品を1個追加する表現ではない。端子自体に増幅・遮断・測定機能を持たない。
      | 端子番号の注意　　　; Connection Portの番号は外箱内の対応番号であり、実パッケージのピン番号とは区別する。
      | 確認の範囲　　　　　; 実ポートと階層対応による静的接続の説明。電気特性の再現性は所属部品の説明を参照する。
      | 
      | 従来の補足　　　　　; 以前のDescriptionを以下に保持する。
      | Physical U7 pin 24 / GP18
      | 
      | 【この説明欄の略語・記号】
      | 用語1　　　　　　　 ; ADC：Analog-to-Digital Converter（アナログ・デジタル変換器）。測定電圧をデジタル値へ変換する回路。電流や温度も、センサーで電圧へ変換した後に読み取る。
      | 用語2　　　　　　　 ; GPIO：General-Purpose Input/Output（汎用入出力端子）。入力・出力や周辺機能に割り当てられる端子。GPの後の数字はRP2040の端子信号番号で、基板上の物理ピン番号とは別。
      | 用語3　　　　　　　 ; SPI：Serial Peripheral Interface（同期式シリアル通信）。クロックとデータ線を使う通信方式。本回路ではRP2040と外付け測定用ADCの通信に使う。
      | 用語4　　　　　　　 ; SCK：Serial Clock（シリアル通信クロック）。SPIのデータを送り受けするタイミングを定める信号。
  Pin_023 : PMIOPort  Description=|  Port=38  Side=Right  ConnectionType=Connection: foundation.electrical.electrical
      | 識別名　　　　　　　; Pin_023
      | 種別　　　　　　　　; Simscape Connection Port（階層境界の物理端子）
      | 所属部品　　　　　　; U7
      | 配置目的　　　　　　; 内部の電気ノードを、この外箱の外側の対応端子へ引き出す。
      | 対応端子　　　　　　; rconn:3／23番 GND
      | 接続ラベル　　　　　; GND、PROT_RETURN
      | モデルの範囲　　　　; 実部品を1個追加する表現ではない。端子自体に増幅・遮断・測定機能を持たない。
      | 端子番号の注意　　　; Connection Portの番号は外箱内の対応番号であり、実パッケージのピン番号とは区別する。
      | 確認の範囲　　　　　; 実ポートと階層対応による静的接続の説明。電気特性の再現性は所属部品の説明を参照する。
      | 
      | 従来の補足　　　　　; 以前のDescriptionを以下に保持する。
      | Physical U7 pin 23 / GND
      | 
      | 【この説明欄の略語・記号】
      | 用語1　　　　　　　 ; GND：Ground（回路の基準電位・電流帰路）。この図の共通基準。保護接地や大地への接続を意味するとは限らない。
      | 用語2　　　　　　　 ; PROT_RETURN：保護回路の共通帰路。PROTはProtection（保護）、RETURNは帰路。プロトタイプの略ではなく、現回路では共通GNDへつながる。
  Pin_022 : PMIOPort  Description=|  Port=39  Side=Right  ConnectionType=Connection: foundation.electrical.electrical
      | 識別名　　　　　　　; Pin_022
      | 種別　　　　　　　　; Simscape Connection Port（階層境界の物理端子）
      | 所属部品　　　　　　; U7
      | 配置目的　　　　　　; 内部の電気ノードを、この外箱の外側の対応端子へ引き出す。
      | 対応端子　　　　　　; rconn:2／22番 GP17
      | 接続ラベル　　　　　; SPI_CS_N
      | モデルの範囲　　　　; 実部品を1個追加する表現ではない。端子自体に増幅・遮断・測定機能を持たない。
      | 端子番号の注意　　　; Connection Portの番号は外箱内の対応番号であり、実パッケージのピン番号とは区別する。
      | 確認の範囲　　　　　; 実ポートと階層対応による静的接続の説明。電気特性の再現性は所属部品の説明を参照する。
      | 
      | 従来の補足　　　　　; 以前のDescriptionを以下に保持する。
      | Physical U7 pin 22 / GP17
      | 
      | 【この説明欄の略語・記号】
      | 用語1　　　　　　　 ; ADC：Analog-to-Digital Converter（アナログ・デジタル変換器）。測定電圧をデジタル値へ変換する回路。電流や温度も、センサーで電圧へ変換した後に読み取る。
      | 用語2　　　　　　　 ; GPIO：General-Purpose Input/Output（汎用入出力端子）。入力・出力や周辺機能に割り当てられる端子。GPの後の数字はRP2040の端子信号番号で、基板上の物理ピン番号とは別。
      | 用語3　　　　　　　 ; SPI：Serial Peripheral Interface（同期式シリアル通信）。クロックとデータ線を使う通信方式。本回路ではRP2040と外付け測定用ADCの通信に使う。
      | 用語4　　　　　　　 ; CS_N：Chip Select（チップ選択信号）。末尾Nはこの設計でLow有効を表す。Lowにして通信対象のADCを選択する。
  Pin_021 : PMIOPort  Description=|  Port=40  Side=Right  ConnectionType=Connection: foundation.electrical.electrical
      | 識別名　　　　　　　; Pin_021
      | 種別　　　　　　　　; Simscape Connection Port（階層境界の物理端子）
      | 所属部品　　　　　　; U7
      | 配置目的　　　　　　; 内部の電気ノードを、この外箱の外側の対応端子へ引き出す。
      | 対応端子　　　　　　; rconn:1／21番 GP16
      | 接続ラベル　　　　　; SPI_MISO
      | モデルの範囲　　　　; 実部品を1個追加する表現ではない。端子自体に増幅・遮断・測定機能を持たない。
      | 端子番号の注意　　　; Connection Portの番号は外箱内の対応番号であり、実パッケージのピン番号とは区別する。
      | 確認の範囲　　　　　; 実ポートと階層対応による静的接続の説明。電気特性の再現性は所属部品の説明を参照する。
      | 
      | 従来の補足　　　　　; 以前のDescriptionを以下に保持する。
      | Physical U7 pin 21 / GP16
      | 
      | 【この説明欄の略語・記号】
      | 用語1　　　　　　　 ; ADC：Analog-to-Digital Converter（アナログ・デジタル変換器）。測定電圧をデジタル値へ変換する回路。電流や温度も、センサーで電圧へ変換した後に読み取る。
      | 用語2　　　　　　　 ; GPIO：General-Purpose Input/Output（汎用入出力端子）。入力・出力や周辺機能に割り当てられる端子。GPの後の数字はRP2040の端子信号番号で、基板上の物理ピン番号とは別。
      | 用語3　　　　　　　 ; SPI：Serial Peripheral Interface（同期式シリアル通信）。クロックとデータ線を使う通信方式。本回路ではRP2040と外付け測定用ADCの通信に使う。
      | 用語4　　　　　　　 ; MISO：Master In, Slave Out（制御側へ入るSPIデータ線）。この回路ではADCのDOUTからRP2040へ測定値が流れる。名称の主従は通信上の役割を表す。
      | 用語5　　　　　　　 ; DOUT：Data Out（データ出力端子）。ADC側から見た変換結果のデジタルデータ出力。
  Pin_041 : PMIOPort  Description=|  Port=41  Side=Right  ConnectionType=Connection: foundation.electrical.electrical
      | 識別名　　　　　　　; Pin_041
      | 種別　　　　　　　　; Simscape Connection Port（階層境界の物理端子）
      | 所属部品　　　　　　; U7
      | 配置目的　　　　　　; 内部の電気ノードを、この外箱の外側の対応端子へ引き出す。
      | 対応端子　　　　　　; rconn:21／D1番 SWCLK
      | 接続ラベル　　　　　; ラベルなし。接続は実線と境界対応で定義する。
      | モデルの範囲　　　　; 実部品を1個追加する表現ではない。端子自体に増幅・遮断・測定機能を持たない。
      | 端子番号の注意　　　; Connection Portの番号は外箱内の対応番号であり、実パッケージのピン番号とは区別する。
      | 確認の範囲　　　　　; 実ポートと階層対応による静的接続の説明。電気特性の再現性は所属部品の説明を参照する。
      | 
      | 従来の補足　　　　　; 以前のDescriptionを以下に保持する。
      | Physical U7 pin D1 / SWCLK
      | 
      | 【この説明欄の略語・記号】
      | 用語1　　　　　　　 ; SWD：Serial Wire Debug（シリアルデバッグ用接続）。SWCLKはデバッグクロック、SWDIOは双方向デバッグデータ、SWD_GNDはその基準。現回路では未接続の端子がある。
      | 用語2　　　　　　　 ; GND：Ground（回路の基準電位・電流帰路）。この図の共通基準。保護接地や大地への接続を意味するとは限らない。
  Pin_042 : PMIOPort  Description=|  Port=42  Side=Right  ConnectionType=Connection: foundation.electrical.electrical
      | 識別名　　　　　　　; Pin_042
      | 種別　　　　　　　　; Simscape Connection Port（階層境界の物理端子）
      | 所属部品　　　　　　; U7
      | 配置目的　　　　　　; 内部の電気ノードを、この外箱の外側の対応端子へ引き出す。
      | 対応端子　　　　　　; rconn:22／D2番 SWD_GND
      | 接続ラベル　　　　　; ラベルなし。接続は実線と境界対応で定義する。
      | モデルの範囲　　　　; 実部品を1個追加する表現ではない。端子自体に増幅・遮断・測定機能を持たない。
      | 端子番号の注意　　　; Connection Portの番号は外箱内の対応番号であり、実パッケージのピン番号とは区別する。
      | 確認の範囲　　　　　; 実ポートと階層対応による静的接続の説明。電気特性の再現性は所属部品の説明を参照する。
      | 
      | 従来の補足　　　　　; 以前のDescriptionを以下に保持する。
      | Physical U7 pin D2 / SWD_GND
      | 
      | 【この説明欄の略語・記号】
      | 用語1　　　　　　　 ; SWD：Serial Wire Debug（シリアルデバッグ用接続）。SWCLKはデバッグクロック、SWDIOは双方向デバッグデータ、SWD_GNDはその基準。現回路では未接続の端子がある。
      | 用語2　　　　　　　 ; GND：Ground（回路の基準電位・電流帰路）。この図の共通基準。保護接地や大地への接続を意味するとは限らない。
  Pin_043 : PMIOPort  Description=|  Port=43  Side=Right  ConnectionType=Connection: foundation.electrical.electrical
      | 識別名　　　　　　　; Pin_043
      | 種別　　　　　　　　; Simscape Connection Port（階層境界の物理端子）
      | 所属部品　　　　　　; U7
      | 配置目的　　　　　　; 内部の電気ノードを、この外箱の外側の対応端子へ引き出す。
      | 対応端子　　　　　　; rconn:23／D3番 SWDIO
      | 接続ラベル　　　　　; ラベルなし。接続は実線と境界対応で定義する。
      | モデルの範囲　　　　; 実部品を1個追加する表現ではない。端子自体に増幅・遮断・測定機能を持たない。
      | 端子番号の注意　　　; Connection Portの番号は外箱内の対応番号であり、実パッケージのピン番号とは区別する。
      | 確認の範囲　　　　　; 実ポートと階層対応による静的接続の説明。電気特性の再現性は所属部品の説明を参照する。
      | 
      | 従来の補足　　　　　; 以前のDescriptionを以下に保持する。
      | Physical U7 pin D3 / SWDIO
      | 
      | 【この説明欄の略語・記号】
      | 用語1　　　　　　　 ; SWD：Serial Wire Debug（シリアルデバッグ用接続）。SWCLKはデバッグクロック、SWDIOは双方向デバッグデータ、SWD_GNDはその基準。現回路では未接続の端子がある。
      | 用語2　　　　　　　 ; GND：Ground（回路の基準電位・電流帰路）。この図の共通基準。保護接地や大地への接続を意味するとは限らない。

== system solar_pv_protected_c07_circuit/U8 ==
  Pin_001 : PMIOPort  Description=|  Side=Left  ConnectionType=Connection: foundation.electrical.electrical
      | 識別名　　　　　　　; Pin_001
      | 種別　　　　　　　　; Simscape Connection Port（階層境界の物理端子）
      | 所属部品　　　　　　; U8
      | 配置目的　　　　　　; 内部の電気ノードを、この外箱の外側の対応端子へ引き出す。
      | 対応端子　　　　　　; lconn:1／1番 ANODE
      | 接続ラベル　　　　　; ラベルなし。接続は実線と境界対応で定義する。
      | モデルの範囲　　　　; 実部品を1個追加する表現ではない。端子自体に増幅・遮断・測定機能を持たない。
      | 端子番号の注意　　　; Connection Portの番号は外箱内の対応番号であり、実パッケージのピン番号とは区別する。
      | 確認の範囲　　　　　; 実ポートと階層対応による静的接続の説明。電気特性の再現性は所属部品の説明を参照する。
      | 
      | 従来の補足　　　　　; 以前のDescriptionを以下に保持する。
      | Physical U8 pin 1 / ANODE
  Pin_002 : PMIOPort  Description=|  Port=2  Side=Left  ConnectionType=Connection: foundation.electrical.electrical
      | 識別名　　　　　　　; Pin_002
      | 種別　　　　　　　　; Simscape Connection Port（階層境界の物理端子）
      | 所属部品　　　　　　; U8
      | 配置目的　　　　　　; 内部の電気ノードを、この外箱の外側の対応端子へ引き出す。
      | 対応端子　　　　　　; lconn:2／2番 NC
      | 接続ラベル　　　　　; ラベルなし。接続は実線と境界対応で定義する。
      | モデルの範囲　　　　; 実部品を1個追加する表現ではない。端子自体に増幅・遮断・測定機能を持たない。
      | 端子番号の注意　　　; Connection Portの番号は外箱内の対応番号であり、実パッケージのピン番号とは区別する。
      | 確認の範囲　　　　　; 実ポートと階層対応による静的接続の説明。電気特性の再現性は所属部品の説明を参照する。
      | 
      | 従来の補足　　　　　; 以前のDescriptionを以下に保持する。
      | Physical U8 pin 2 / NC
      | 
      | 【この説明欄の略語・記号】
      | 用語1　　　　　　　 ; NC：No Connection（接続しない端子）。メーカー指定の未接続端子。一般の使用していない信号端子と同一に扱わない。
  Pin_003 : PMIOPort  Description=|  Port=3  Side=Left  ConnectionType=Connection: foundation.electrical.electrical
      | 識別名　　　　　　　; Pin_003
      | 種別　　　　　　　　; Simscape Connection Port（階層境界の物理端子）
      | 所属部品　　　　　　; U8
      | 配置目的　　　　　　; 内部の電気ノードを、この外箱の外側の対応端子へ引き出す。
      | 対応端子　　　　　　; lconn:3／3番 CATHODE
      | 接続ラベル　　　　　; ラベルなし。接続は実線と境界対応で定義する。
      | モデルの範囲　　　　; 実部品を1個追加する表現ではない。端子自体に増幅・遮断・測定機能を持たない。
      | 端子番号の注意　　　; Connection Portの番号は外箱内の対応番号であり、実パッケージのピン番号とは区別する。
      | 確認の範囲　　　　　; 実ポートと階層対応による静的接続の説明。電気特性の再現性は所属部品の説明を参照する。
      | 
      | 従来の補足　　　　　; 以前のDescriptionを以下に保持する。
      | Physical U8 pin 3 / CATHODE
  Pin_006 : PMIOPort  Description=|  Port=4  Side=Right  ConnectionType=Connection: foundation.electrical.electrical
      | 識別名　　　　　　　; Pin_006
      | 種別　　　　　　　　; Simscape Connection Port（階層境界の物理端子）
      | 所属部品　　　　　　; U8
      | 配置目的　　　　　　; 内部の電気ノードを、この外箱の外側の対応端子へ引き出す。
      | 対応端子　　　　　　; rconn:3／6番 VCC
      | 接続ラベル　　　　　; H12
      | モデルの範囲　　　　; 実部品を1個追加する表現ではない。端子自体に増幅・遮断・測定機能を持たない。
      | 端子番号の注意　　　; Connection Portの番号は外箱内の対応番号であり、実パッケージのピン番号とは区別する。
      | 確認の範囲　　　　　; 実ポートと階層対応による静的接続の説明。電気特性の再現性は所属部品の説明を参照する。
      | 
      | 従来の補足　　　　　; 以前のDescriptionを以下に保持する。
      | Physical U8 pin 6 / VCC
      | 
      | 【この説明欄の略語・記号】
      | 用語1　　　　　　　 ; IC：Integrated Circuit（集積回路）。複数の電子素子と機能を小さな半導体チップに集積した部品。
      | 用語2　　　　　　　 ; MOSFET：Metal-Oxide-Semiconductor Field-Effect Transistor（金属・酸化膜・半導体構造の電界効果トランジスタ）。ゲートとソースの電圧でドレインとソースの導通を制御する素子。N-MOSはNチャネル型を表す。
      | 用語3　　　　　　　 ; GND：Ground（回路の基準電位・電流帰路）。この図の共通基準。保護接地や大地への接続を意味するとは限らない。
      | 用語4　　　　　　　 ; VCC/VDD/VEE/VS：ICの電源端子名。文字の歴史的な由来を現在の接続機能へ当てはめない。現回路のVEEはU8/U10では浮動基準SW、U9ではGND。各電圧・基準は端子と接続を参照する。
      | 用語5　　　　　　　 ; SW：Switching Node（スイッチング点）。主電力段の上下MOSFETとL1がつながる、電圧が高速に切り替わる点。GNDとは別電位。
  Pin_005 : PMIOPort  Description=|  Port=5  Side=Right  ConnectionType=Connection: foundation.electrical.electrical
      | 識別名　　　　　　　; Pin_005
      | 種別　　　　　　　　; Simscape Connection Port（階層境界の物理端子）
      | 所属部品　　　　　　; U8
      | 配置目的　　　　　　; 内部の電気ノードを、この外箱の外側の対応端子へ引き出す。
      | 対応端子　　　　　　; rconn:2／5番 VOUT
      | 接続ラベル　　　　　; ラベルなし。接続は実線と境界対応で定義する。
      | モデルの範囲　　　　; 実部品を1個追加する表現ではない。端子自体に増幅・遮断・測定機能を持たない。
      | 端子番号の注意　　　; Connection Portの番号は外箱内の対応番号であり、実パッケージのピン番号とは区別する。
      | 確認の範囲　　　　　; 実ポートと階層対応による静的接続の説明。電気特性の再現性は所属部品の説明を参照する。
      | 
      | 従来の補足　　　　　; 以前のDescriptionを以下に保持する。
      | Physical U8 pin 5 / VOUT
      | 
      | 【この説明欄の略語・記号】
      | 用語1　　　　　　　 ; VIN/VOUT：入力電圧・出力電圧を表す端子／ネット名。INは入力、OUTは出力。電源変換器の電力端子なのか、検出用端子なのかは対象部品によって異なるため、端子と接続の説明に従う。
  Pin_004 : PMIOPort  Description=|  Port=6  Side=Right  ConnectionType=Connection: foundation.electrical.electrical
      | 識別名　　　　　　　; Pin_004
      | 種別　　　　　　　　; Simscape Connection Port（階層境界の物理端子）
      | 所属部品　　　　　　; U8
      | 配置目的　　　　　　; 内部の電気ノードを、この外箱の外側の対応端子へ引き出す。
      | 対応端子　　　　　　; rconn:1／4番 VEE
      | 接続ラベル　　　　　; ラベルなし。接続は実線と境界対応で定義する。
      | モデルの範囲　　　　; 実部品を1個追加する表現ではない。端子自体に増幅・遮断・測定機能を持たない。
      | 端子番号の注意　　　; Connection Portの番号は外箱内の対応番号であり、実パッケージのピン番号とは区別する。
      | 確認の範囲　　　　　; 実ポートと階層対応による静的接続の説明。電気特性の再現性は所属部品の説明を参照する。
      | 
      | 従来の補足　　　　　; 以前のDescriptionを以下に保持する。
      | Physical U8 pin 4 / VEE
      | 
      | 【この説明欄の略語・記号】
      | 用語1　　　　　　　 ; IC：Integrated Circuit（集積回路）。複数の電子素子と機能を小さな半導体チップに集積した部品。
      | 用語2　　　　　　　 ; MOSFET：Metal-Oxide-Semiconductor Field-Effect Transistor（金属・酸化膜・半導体構造の電界効果トランジスタ）。ゲートとソースの電圧でドレインとソースの導通を制御する素子。N-MOSはNチャネル型を表す。
      | 用語3　　　　　　　 ; GND：Ground（回路の基準電位・電流帰路）。この図の共通基準。保護接地や大地への接続を意味するとは限らない。
      | 用語4　　　　　　　 ; VCC/VDD/VEE/VS：ICの電源端子名。文字の歴史的な由来を現在の接続機能へ当てはめない。現回路のVEEはU8/U10では浮動基準SW、U9ではGND。各電圧・基準は端子と接続を参照する。
      | 用語5　　　　　　　 ; SW：Switching Node（スイッチング点）。主電力段の上下MOSFETとL1がつながる、電圧が高速に切り替わる点。GNDとは別電位。

== system solar_pv_protected_c07_circuit/U9 ==
  Pin_001 : PMIOPort  Description=|  Side=Left  ConnectionType=Connection: foundation.electrical.electrical
      | 識別名　　　　　　　; Pin_001
      | 種別　　　　　　　　; Simscape Connection Port（階層境界の物理端子）
      | 所属部品　　　　　　; U9
      | 配置目的　　　　　　; 内部の電気ノードを、この外箱の外側の対応端子へ引き出す。
      | 対応端子　　　　　　; lconn:1／1番 ANODE
      | 接続ラベル　　　　　; ラベルなし。接続は実線と境界対応で定義する。
      | モデルの範囲　　　　; 実部品を1個追加する表現ではない。端子自体に増幅・遮断・測定機能を持たない。
      | 端子番号の注意　　　; Connection Portの番号は外箱内の対応番号であり、実パッケージのピン番号とは区別する。
      | 確認の範囲　　　　　; 実ポートと階層対応による静的接続の説明。電気特性の再現性は所属部品の説明を参照する。
      | 
      | 従来の補足　　　　　; 以前のDescriptionを以下に保持する。
      | Physical U9 pin 1 / ANODE
  Pin_002 : PMIOPort  Description=|  Port=2  Side=Left  ConnectionType=Connection: foundation.electrical.electrical
      | 識別名　　　　　　　; Pin_002
      | 種別　　　　　　　　; Simscape Connection Port（階層境界の物理端子）
      | 所属部品　　　　　　; U9
      | 配置目的　　　　　　; 内部の電気ノードを、この外箱の外側の対応端子へ引き出す。
      | 対応端子　　　　　　; lconn:2／2番 NC
      | 接続ラベル　　　　　; ラベルなし。接続は実線と境界対応で定義する。
      | モデルの範囲　　　　; 実部品を1個追加する表現ではない。端子自体に増幅・遮断・測定機能を持たない。
      | 端子番号の注意　　　; Connection Portの番号は外箱内の対応番号であり、実パッケージのピン番号とは区別する。
      | 確認の範囲　　　　　; 実ポートと階層対応による静的接続の説明。電気特性の再現性は所属部品の説明を参照する。
      | 
      | 従来の補足　　　　　; 以前のDescriptionを以下に保持する。
      | Physical U9 pin 2 / NC
      | 
      | 【この説明欄の略語・記号】
      | 用語1　　　　　　　 ; NC：No Connection（接続しない端子）。メーカー指定の未接続端子。一般の使用していない信号端子と同一に扱わない。
  Pin_003 : PMIOPort  Description=|  Port=3  Side=Left  ConnectionType=Connection: foundation.electrical.electrical
      | 識別名　　　　　　　; Pin_003
      | 種別　　　　　　　　; Simscape Connection Port（階層境界の物理端子）
      | 所属部品　　　　　　; U9
      | 配置目的　　　　　　; 内部の電気ノードを、この外箱の外側の対応端子へ引き出す。
      | 対応端子　　　　　　; lconn:3／3番 CATHODE
      | 接続ラベル　　　　　; ラベルなし。接続は実線と境界対応で定義する。
      | モデルの範囲　　　　; 実部品を1個追加する表現ではない。端子自体に増幅・遮断・測定機能を持たない。
      | 端子番号の注意　　　; Connection Portの番号は外箱内の対応番号であり、実パッケージのピン番号とは区別する。
      | 確認の範囲　　　　　; 実ポートと階層対応による静的接続の説明。電気特性の再現性は所属部品の説明を参照する。
      | 
      | 従来の補足　　　　　; 以前のDescriptionを以下に保持する。
      | Physical U9 pin 3 / CATHODE
  Pin_006 : PMIOPort  Description=|  Port=4  Side=Right  ConnectionType=Connection: foundation.electrical.electrical
      | 識別名　　　　　　　; Pin_006
      | 種別　　　　　　　　; Simscape Connection Port（階層境界の物理端子）
      | 所属部品　　　　　　; U9
      | 配置目的　　　　　　; 内部の電気ノードを、この外箱の外側の対応端子へ引き出す。
      | 対応端子　　　　　　; rconn:3／6番 VCC
      | 接続ラベル　　　　　; P12
      | モデルの範囲　　　　; 実部品を1個追加する表現ではない。端子自体に増幅・遮断・測定機能を持たない。
      | 端子番号の注意　　　; Connection Portの番号は外箱内の対応番号であり、実パッケージのピン番号とは区別する。
      | 確認の範囲　　　　　; 実ポートと階層対応による静的接続の説明。電気特性の再現性は所属部品の説明を参照する。
      | 
      | 従来の補足　　　　　; 以前のDescriptionを以下に保持する。
      | Physical U9 pin 6 / VCC
      | 
      | 【この説明欄の略語・記号】
      | 用語1　　　　　　　 ; IC：Integrated Circuit（集積回路）。複数の電子素子と機能を小さな半導体チップに集積した部品。
      | 用語2　　　　　　　 ; MOSFET：Metal-Oxide-Semiconductor Field-Effect Transistor（金属・酸化膜・半導体構造の電界効果トランジスタ）。ゲートとソースの電圧でドレインとソースの導通を制御する素子。N-MOSはNチャネル型を表す。
      | 用語3　　　　　　　 ; GND：Ground（回路の基準電位・電流帰路）。この図の共通基準。保護接地や大地への接続を意味するとは限らない。
      | 用語4　　　　　　　 ; VCC/VDD/VEE/VS：ICの電源端子名。文字の歴史的な由来を現在の接続機能へ当てはめない。現回路のVEEはU8/U10では浮動基準SW、U9ではGND。各電圧・基準は端子と接続を参照する。
      | 用語5　　　　　　　 ; SW：Switching Node（スイッチング点）。主電力段の上下MOSFETとL1がつながる、電圧が高速に切り替わる点。GNDとは別電位。
  Pin_005 : PMIOPort  Description=|  Port=5  Side=Right  ConnectionType=Connection: foundation.electrical.electrical
      | 識別名　　　　　　　; Pin_005
      | 種別　　　　　　　　; Simscape Connection Port（階層境界の物理端子）
      | 所属部品　　　　　　; U9
      | 配置目的　　　　　　; 内部の電気ノードを、この外箱の外側の対応端子へ引き出す。
      | 対応端子　　　　　　; rconn:2／5番 VOUT
      | 接続ラベル　　　　　; ラベルなし。接続は実線と境界対応で定義する。
      | モデルの範囲　　　　; 実部品を1個追加する表現ではない。端子自体に増幅・遮断・測定機能を持たない。
      | 端子番号の注意　　　; Connection Portの番号は外箱内の対応番号であり、実パッケージのピン番号とは区別する。
      | 確認の範囲　　　　　; 実ポートと階層対応による静的接続の説明。電気特性の再現性は所属部品の説明を参照する。
      | 
      | 従来の補足　　　　　; 以前のDescriptionを以下に保持する。
      | Physical U9 pin 5 / VOUT
      | 
      | 【この説明欄の略語・記号】
      | 用語1　　　　　　　 ; VIN/VOUT：入力電圧・出力電圧を表す端子／ネット名。INは入力、OUTは出力。電源変換器の電力端子なのか、検出用端子なのかは対象部品によって異なるため、端子と接続の説明に従う。
  Pin_004 : PMIOPort  Description=|  Port=6  Side=Right  ConnectionType=Connection: foundation.electrical.electrical
      | 識別名　　　　　　　; Pin_004
      | 種別　　　　　　　　; Simscape Connection Port（階層境界の物理端子）
      | 所属部品　　　　　　; U9
      | 配置目的　　　　　　; 内部の電気ノードを、この外箱の外側の対応端子へ引き出す。
      | 対応端子　　　　　　; rconn:1／4番 VEE
      | 接続ラベル　　　　　; GND、PROT_RETURN
      | モデルの範囲　　　　; 実部品を1個追加する表現ではない。端子自体に増幅・遮断・測定機能を持たない。
      | 端子番号の注意　　　; Connection Portの番号は外箱内の対応番号であり、実パッケージのピン番号とは区別する。
      | 確認の範囲　　　　　; 実ポートと階層対応による静的接続の説明。電気特性の再現性は所属部品の説明を参照する。
      | 
      | 従来の補足　　　　　; 以前のDescriptionを以下に保持する。
      | Physical U9 pin 4 / VEE
      | 
      | 【この説明欄の略語・記号】
      | 用語1　　　　　　　 ; IC：Integrated Circuit（集積回路）。複数の電子素子と機能を小さな半導体チップに集積した部品。
      | 用語2　　　　　　　 ; MOSFET：Metal-Oxide-Semiconductor Field-Effect Transistor（金属・酸化膜・半導体構造の電界効果トランジスタ）。ゲートとソースの電圧でドレインとソースの導通を制御する素子。N-MOSはNチャネル型を表す。
      | 用語3　　　　　　　 ; GND：Ground（回路の基準電位・電流帰路）。この図の共通基準。保護接地や大地への接続を意味するとは限らない。
      | 用語4　　　　　　　 ; VCC/VDD/VEE/VS：ICの電源端子名。文字の歴史的な由来を現在の接続機能へ当てはめない。現回路のVEEはU8/U10では浮動基準SW、U9ではGND。各電圧・基準は端子と接続を参照する。
      | 用語5　　　　　　　 ; SW：Switching Node（スイッチング点）。主電力段の上下MOSFETとL1がつながる、電圧が高速に切り替わる点。GNDとは別電位。
      | 用語6　　　　　　　 ; PROT_RETURN：保護回路の共通帰路。PROTはProtection（保護）、RETURNは帰路。プロトタイプの略ではなく、現回路では共通GNDへつながる。
